simulink library "ride_lib"  (R2025b)
settings: Solver=VariableStepAuto  StartTime=0.0  StopTime=10.0  RelTol=1e-3
undefined symbols (not defined in the file or in its folder): ride
libraries: $bdroot x3
settings Model: Creator=mohammedazab  LastModifiedBy=mohammedazab

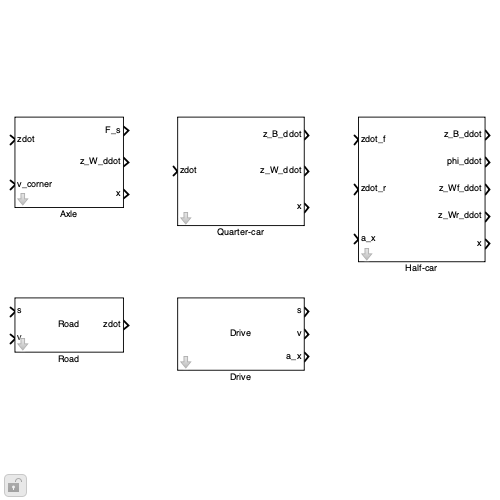
[thumbnail: Simulink's stored preview of the top-level diagram]
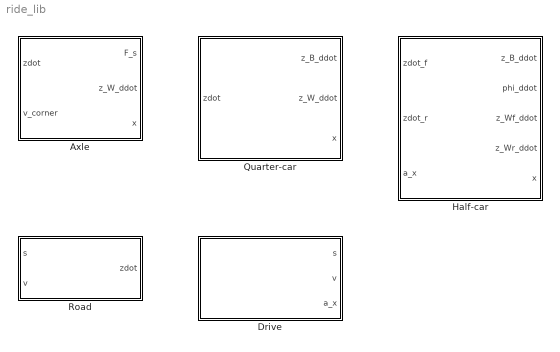
== system ride_lib ==
  Axle : Subsystem  mask(Axle){m_W=50.399999999999999, k_T=262200, c_T=500, k_S=27922, dz_S_stat=0.16361711195473103, dz_cmp=0.02, dz_rbd=0.080000000000000002, f1_cmp=0.33333333329999998, f2_cmp=4, f1_rbd=1, f2_rbd=8, F_max=100000, D=3530, A=0.5, v_d=0.20000000000000001, v_z=0.20000000000000001}
      mask prompts: m_W "Wheel mass m_W [kg]"; k_T "Tyre stiffness k_T [N/m]"; c_T "Tyre damping c_T [N s/m]"; k_S "Spring stiffness k_S [N/m]"; dz_S_stat "Static spring deflection dz_S_stat [m]"; dz_cmp "Compression knee dz_cmp [m]"; dz_rbd "Rebound knee dz_rbd [m]"; f1_cmp "Compression shape f1_cmp [-]"; f2_cmp "Compression rate f2_cmp [-]"; f1_rbd "Rebound shape f1_rbd [-]"; f2_rbd "Rebound rate f2_rbd [-]"; F_max "Spring force limit F_max [N]"; D "Damper coefficient D [N s/m]"; A "Damper asymmetry A [-]"; v_d "Compression knee velocity v_d [m/s]"; v_z "Rebound knee velocity v_z [m/s]"
      mask help: One axle: tyre spring and damper, wheel mass, progressive suspension spring and asymmetric damper. F_s is the suspension force on the body, positive upward. x = [tyre deflection; wheel velocity; suspension deflection].
      mask init:
      | c = ride.core.suspension.damper_coefficients(D, A); d1 = c.d1; z1 = c.z1; d2 = c.d2; z2 = c.z2;
      mask Display:
      | port_label('input', 1, 'zdot');
      | port_label('input', 2, 'v_corner');
      | port_label('output', 1, 'F_s');
      | port_label('output', 2, 'z_W_ddot');
      | port_label('output', 3, 'x');
  Drive : Subsystem  mask(Drive){speeds=6 * ones(500, 1), dt=0.02}
      mask prompts: speeds "Speed at every step [m/s]"; dt "Step dt [s]"
      mask help: Speed profile played back in steps of dt: speed v [m/s] held over each step, distance s [m] and the longitudinal acceleration a_x = (v_k - v_(k-1)) / dt [m/s^2], as in ride.simulate.
      mask init:
      | speed_table = [(0:numel(speeds) - 1)' * dt, speeds(:)];
      mask Display:
      | disp('Drive');
      | port_label('output', 1, 's');
      | port_label('output', 2, 'v');
      | port_label('output', 3, 'a_x');
  Half-car : Subsystem  mask(Half-car){m_B=803, I_B=1430, l_f=1.206, l_r=1.6639999999999999, h_T=0.59999999999999998, h_B=0.222, front_m_W=50.399999999999999, front_k_T=262200, front_c_T=500, front_k_S=29589.900000000001, front_dz_S_stat=0.16361320259798129, front_dz_cmp=0.02, front_dz_rbd=0.080000000000000002, front_f1_cmp=0.33333333329999998, front_f2_cmp=4, front_f1_rbd=1, front_f2_rbd=8, front_F_max=100000, front_D=564.80000000000007, front_A=0.5, front_v_d=0.20000000000000001, front_v_z=0.20000000000000001, rear_m_W=50.399999999999999, rear_k_T=262200, rear_c_T=500, rear_k_S=21444.860000000001, rear_dz_S_stat=0.16361857789913259, rear_dz_cmp=0.02, rear_dz_rbd=0.080000000000000002, rear_f1_cmp=0.33333333329999998, rear_f2_cmp=4, rear_f1_rbd=1, rear_f2_rbd=8, rear_F_max=100000, rear_D=562.39999999999998, rear_A=0.5, rear_v_d=0.20000000000000001, rear_v_z=0.20000000000000001}
      mask prompts: m_B "Body mass m_B [kg]"; I_B "Pitch inertia I_B [kg m^2]"; l_f "Centre of mass to front axle l_f [m]"; l_r "Centre of mass to rear axle l_r [m]"; h_T "Pitch centre height under traction h_T [m]"; h_B "Pitch centre height under braking h_B [m]"; front_m_W "Wheel mass m_W [kg]"; front_k_T "Tyre stiffness k_T [N/m]"; front_c_T "Tyre damping c_T [N s/m]"; front_k_S "Spring stiffness k_S [N/m]"; front_dz_S_stat "Static spring deflection dz_S_stat [m]"; front_dz_cmp "Compression knee dz_cmp [m]"; front_dz_rbd "Rebound knee dz_rbd [m]"; front_f1_cmp "Compression shape f1_cmp [-]"; front_f2_cmp "Compression rate f2_cmp [-]"; front_f1_rbd "Rebound shape f1_rbd [-]"; front_f2_rbd "Rebound rate f2_rbd [-]"; front_F_max "Spring force limit F_max [N]"; front_D "Damper coefficient D [N s/m]"; front_A "Damper asymmetry A [-]"; front_v_d "Compression knee velocity v_d [m/s]"; front_v_z "Rebound knee velocity v_z [m/s]"; rear_m_W "Wheel mass m_W [kg]"; rear_k_T "Tyre stiffness k_T [N/m]"; rear_c_T "Tyre damping c_T [N s/m]"; rear_k_S "Spring stiffness k_S [N/m]"; rear_dz_S_stat "Static spring deflection dz_S_stat [m]"; rear_dz_cmp "Compression knee dz_cmp [m]"; rear_dz_rbd "Rebound knee dz_rbd [m]"; rear_f1_cmp "Compression shape f1_cmp [-]"; rear_f2_cmp "Compression rate f2_cmp [-]"; rear_f1_rbd "Rebound shape f1_rbd [-]"; rear_f2_rbd "Rebound rate f2_rbd [-]"; rear_F_max "Spring force limit F_max [N]"; rear_D "Damper coefficient D [N s/m]"; rear_A "Damper asymmetry A [-]"; rear_v_d "Compression knee velocity v_d [m/s]"; rear_v_z "Rebound knee velocity v_z [m/s]"
      mask help: Half-car ride model: two axles, body heave and pitch, load transfer from the longitudinal acceleration a_x (pitch centre at h_T when a_x > 0, at h_B otherwise). Inputs: road height rate under the front and the rear wheel [m/s] and a_x [m/s^2]. Outputs: body heave and pitch acceleration, front and rear wheel acceleration, and x = [rear tyre deflection; rear wheel velocity; rear suspension deflection; front tyre deflection; front wheel velocity; front suspension deflection; body velocity; pitch rate; body position; pitch angle]. Defaults come from data/models/halfcar/params.json.
      mask init:
      | m_tot = m_B + front_m_W + rear_m_W;
      mask DialogControl body_group Prompt: Body
      mask DialogControl front_group Prompt: Front axle
      mask DialogControl rear_group Prompt: Rear axle
      mask Display:
      | port_label('input', 1, 'zdot_f');
      | port_label('input', 2, 'zdot_r');
      | port_label('input', 3, 'a_x');
      | port_label('output', 1, 'z_B_ddot');
      | port_label('output', 2, 'phi_ddot');
      | port_label('output', 3, 'z_Wf_ddot');
      | port_label('output', 4, 'z_Wr_ddot');
      | port_label('output', 5, 'x');
  Quarter-car : Subsystem  mask(Quarter-car){m_B=465.69999999999999, m_W=50.399999999999999, k_T=262200, c_T=500, k_S=27922, dz_S_stat=0.16361711195473103, dz_cmp=0.02, dz_rbd=0.080000000000000002, f1_cmp=0.33333333329999998, f2_cmp=4, f1_rbd=1, f2_rbd=8, F_max=100000, D=3530, A=0.5, v_d=0.20000000000000001, v_z=0.20000000000000001}
      mask prompts: m_B "Body mass m_B [kg]"; m_W "Wheel mass m_W [kg]"; k_T "Tyre stiffness k_T [N/m]"; c_T "Tyre damping c_T [N s/m]"; k_S "Spring stiffness k_S [N/m]"; dz_S_stat "Static spring deflection dz_S_stat [m]"; dz_cmp "Compression knee dz_cmp [m]"; dz_rbd "Rebound knee dz_rbd [m]"; f1_cmp "Compression shape f1_cmp [-]"; f2_cmp "Compression rate f2_cmp [-]"; f1_rbd "Rebound shape f1_rbd [-]"; f2_rbd "Rebound rate f2_rbd [-]"; F_max "Spring force limit F_max [N]"; D "Damper coefficient D [N s/m]"; A "Damper asymmetry A [-]"; v_d "Compression knee velocity v_d [m/s]"; v_z "Rebound knee velocity v_z [m/s]"
      mask help: Quarter-car ride model: one axle under a quarter of the body, heave only. Input: road height rate under the wheel [m/s]. Outputs: body and wheel vertical acceleration [m/s^2] and the states x = [tyre deflection; wheel velocity; suspension deflection; body velocity; body position]. Defaults come from data/models/quartercar/params.json.
      mask DialogControl body_group Prompt: Body
      mask DialogControl axle_group Prompt: Axle
      mask Display:
      | port_label('input', 1, 'zdot');
      | port_label('output', 1, 'z_B_ddot');
      | port_label('output', 2, 'z_W_ddot');
      | port_label('output', 3, 'x');
  Road : Subsystem  mask(Road){road=ride.core.terrain.bumps([20 0.06 2]), lag_m=0}
      mask prompts: road "Terrain struct (scenario.road)"; lag_m "Distance behind the front axle [m]"
      mask help: Road height rate under a wheel that runs lag_m behind the front axle. road is a terrain struct from ride.core.terrain (a scenario's road field): a bump list or a measured profile.
      mask init:
      | lag = lag_m;
      | if strcmp(road.type, 'profile')
      |     kind = 2; ds = road.ds; dz = road.dz(:); bumps = zeros(1, 3);
      | else
      |     kind = 1; ds = 1; dz = zeros(2, 1); bumps = road.bumps;
      |     if isempty(bumps)
      |         bumps = zeros(1, 3);
      |     end
      | end
      mask Display:
      | disp('Road');
      | port_label('input', 1, 's');
      | port_label('input', 2, 'v');
      | port_label('output', 1, 'zdot');

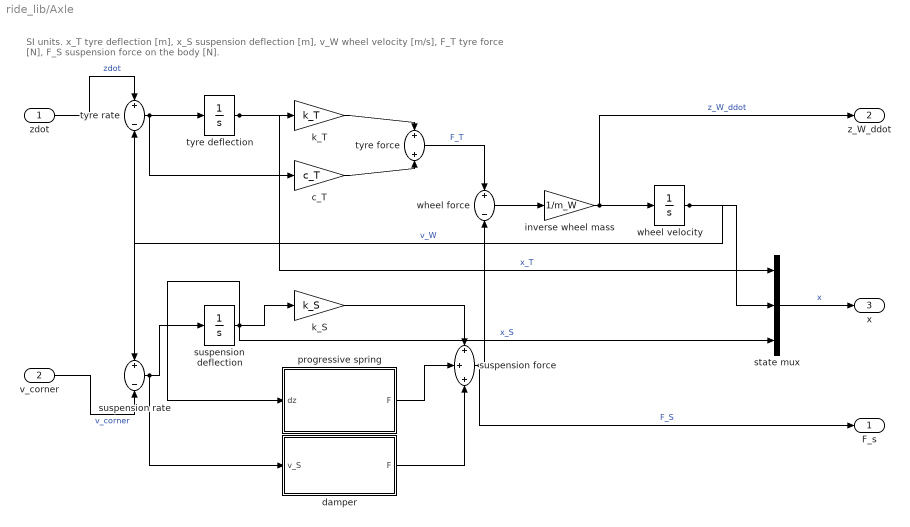
== system ride_lib/Axle ==
  note: SI units. x_T tyre deflection [m], x_S suspension deflection [m], v_W wheel velocity [m/s], F_T tyre force [N], F_S suspension force on the body [N].
  zdot : Inport
  v_corner : Inport  Port=2
  c_T : Gain  Gain=c_T
  damper : MATLAB Function  TreatAsAtomicUnit=on
  inverse wheel mass : Gain  Gain=1/m_W
  k_S : Gain  Gain=k_S
  k_T : Gain  Gain=k_T
  progressive spring : MATLAB Function  TreatAsAtomicUnit=on
  state mux : Mux  Inputs=3
  suspension deflection : Integrator
  suspension force : Sum  Inputs=+++
  suspension rate : Sum  Inputs=+-
  tyre deflection : Integrator
  tyre force : Sum
  tyre rate : Sum  Inputs=+-
  wheel force : Sum  Inputs=+-
  wheel velocity : Integrator
  F_s : Outport
  z_W_ddot : Outport  Port=2
  x : Outport  Port=3
  wires:
  zdot/1 -> tyre rate/1  "zdot"
  wheel velocity/1 -> tyre rate/2, suspension rate/1, state mux/2  "v_W"
  tyre rate/1 -> tyre deflection/1, c_T/1
  tyre deflection/1 -> k_T/1, state mux/1  "x_T"
  k_T/1 -> tyre force/1
  c_T/1 -> tyre force/2
  tyre force/1 -> wheel force/1  "F_T"
  suspension force/1 -> wheel force/2, F_s/1  "F_S"
  wheel force/1 -> inverse wheel mass/1
  inverse wheel mass/1 -> wheel velocity/1, z_W_ddot/1  "z_W_ddot"
  v_corner/1 -> suspension rate/2  "v_corner"
  suspension rate/1 -> suspension deflection/1, damper/1(v_S)
  suspension deflection/1 -> k_S/1, progressive spring/1(dz), state mux/3  "x_S"
  k_S/1 -> suspension force/1
  progressive spring/1(F) -> suspension force/2
  damper/1(F) -> suspension force/3
  state mux/1 -> x/1  "x"

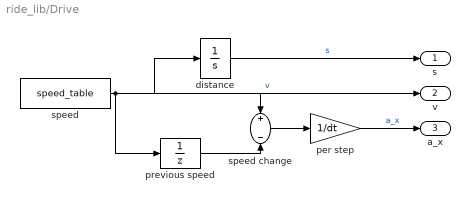
== system ride_lib/Drive ==
  distance : Integrator
  per step : Gain  Gain=1/dt
  previous speed : UnitDelay  InitialCondition=speeds(1)  SampleTime=dt  HasFrameUpgradeWarning=on
  speed : FromWorkspace  VariableName=speed_table  SampleTime=dt  Interpolate=off  OutputAfterFinalValue=Holding final value
  speed change : Sum  Inputs=+-
  s : Outport
  v : Outport  Port=2
  a_x : Outport  Port=3
  wires:
  speed/1 -> distance/1, v/1, speed change/1, previous speed/1  "v"
  distance/1 -> s/1  "s"
  previous speed/1 -> speed change/2
  speed change/1 -> per step/1
  per step/1 -> a_x/1  "a_x"

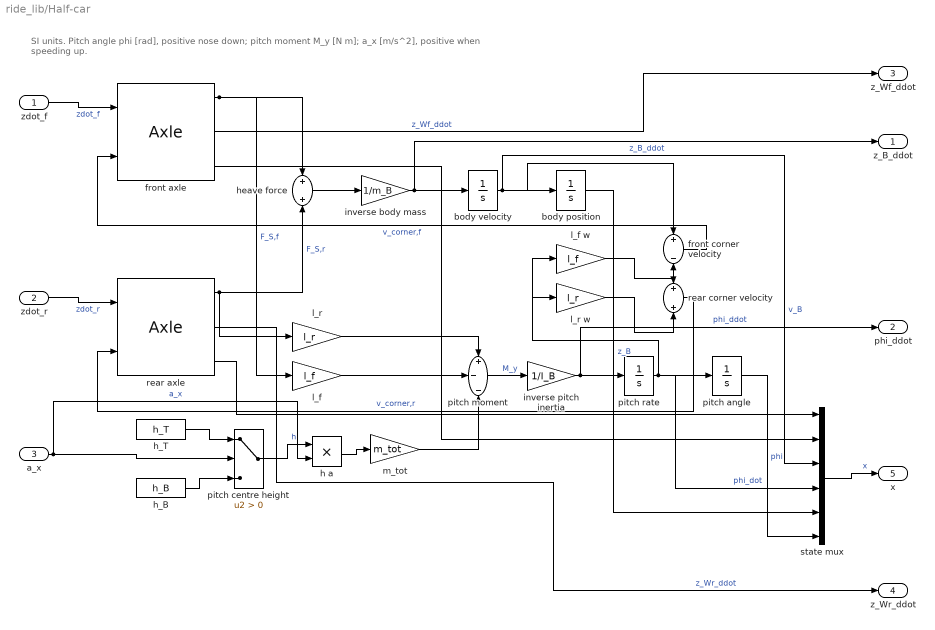
== system ride_lib/Half-car ==
  note: SI units. Pitch angle phi [rad], positive nose down; pitch moment M_y [N m]; a_x [m/s^2], positive when speeding up.
  zdot_f : Inport
  zdot_r : Inport  Port=2
  a_x : Inport  Port=3
  body position : Integrator
  body velocity : Integrator
  front axle : $bdroot/Axle  m_W=front_m_W  k_T=front_k_T  c_T=front_c_T  k_S=front_k_S  dz_S_stat=front_dz_S_stat  dz_cmp=front_dz_cmp  dz_rbd=front_dz_rbd  f1_cmp=front_f1_cmp  f2_cmp=front_f2_cmp  f1_rbd=front_f1_rbd  f2_rbd=front_f2_rbd  F_max=front_F_max  D=front_D  A=front_A  v_d=front_v_d  v_z=front_v_z
  front corner velocity : Sum  Inputs=+-
  h a : Product
  h_B : Constant  Value=h_B
  h_T : Constant  Value=h_T
  heave force : Sum
  inverse body mass : Gain  Gain=1/m_B
  inverse pitch inertia : Gain  Gain=1/I_B
  l_f : Gain  Gain=l_f
  l_f w : Gain  Gain=l_f
  l_r : Gain  Gain=l_r
  l_r w : Gain  Gain=l_r
  m_tot : Gain  Gain=m_tot
  pitch angle : Integrator
  pitch centre height : Switch  Criteria=u2 > Threshold  SaturateOnIntegerOverflow=off  InputSameDT=off
  pitch moment : Sum  Inputs=+--
  pitch rate : Integrator
  rear axle : $bdroot/Axle  m_W=rear_m_W  k_T=rear_k_T  c_T=rear_c_T  k_S=rear_k_S  dz_S_stat=rear_dz_S_stat  dz_cmp=rear_dz_cmp  dz_rbd=rear_dz_rbd  f1_cmp=rear_f1_cmp  f2_cmp=rear_f2_cmp  f1_rbd=rear_f1_rbd  f2_rbd=rear_f2_rbd  F_max=rear_F_max  D=rear_D  A=rear_A  v_d=rear_v_d  v_z=rear_v_z
  rear corner velocity : Sum
  state mux : Mux  Inputs=[3 3 1 1 1 1]
  z_B_ddot : Outport
  phi_ddot : Outport  Port=2
  z_Wf_ddot : Outport  Port=3
  z_Wr_ddot : Outport  Port=4
  x : Outport  Port=5
  wires:
  zdot_f/1 -> front axle/1  "zdot_f"
  zdot_r/1 -> rear axle/1  "zdot_r"
  front corner velocity/1 -> front axle/2  "v_corner,f"
  rear corner velocity/1 -> rear axle/2  "v_corner,r"
  front axle/1 -> heave force/1, l_f/1  "F_S,f"
  rear axle/1 -> heave force/2, l_r/1  "F_S,r"
  heave force/1 -> inverse body mass/1
  inverse body mass/1 -> body velocity/1, z_B_ddot/1  "z_B_ddot"
  body velocity/1 -> body position/1, front corner velocity/1, rear corner velocity/1, state mux/3  "v_B"
  h_T/1 -> pitch centre height/1
  a_x/1 -> pitch centre height/2, h a/2  "a_x"
  h_B/1 -> pitch centre height/3
  pitch centre height/1 -> h a/1  "h"
  h a/1 -> m_tot/1
  l_r/1 -> pitch moment/1
  l_f/1 -> pitch moment/2
  m_tot/1 -> pitch moment/3
  pitch moment/1 -> inverse pitch inertia/1  "M_y"
  inverse pitch inertia/1 -> pitch rate/1, phi_ddot/1  "phi_ddot"
  pitch rate/1 -> pitch angle/1, l_f w/1, l_r w/1, state mux/4  "phi_dot"
  l_f w/1 -> front corner velocity/2
  l_r w/1 -> rear corner velocity/2
  front axle/2 -> z_Wf_ddot/1  "z_Wf_ddot"
  rear axle/2 -> z_Wr_ddot/1  "z_Wr_ddot"
  rear axle/3 -> state mux/1
  front axle/3 -> state mux/2
  body position/1 -> state mux/5  "z_B"
  pitch angle/1 -> state mux/6  "phi"
  state mux/1 -> x/1  "x"

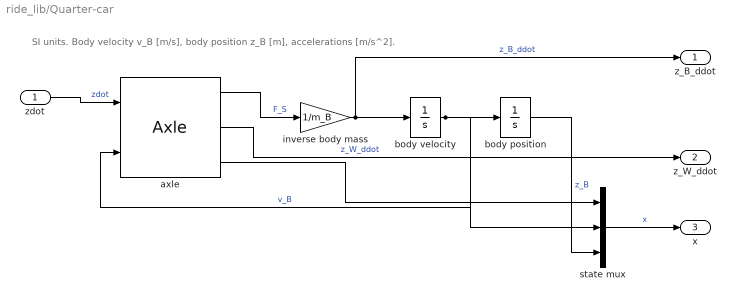
== system ride_lib/Quarter-car ==
  note: SI units. Body velocity v_B [m/s], body position z_B [m], accelerations [m/s^2].
  zdot : Inport
  axle : $bdroot/Axle  m_W=m_W  k_T=k_T  c_T=c_T  k_S=k_S  dz_S_stat=dz_S_stat  dz_cmp=dz_cmp  dz_rbd=dz_rbd  f1_cmp=f1_cmp  f2_cmp=f2_cmp  f1_rbd=f1_rbd  f2_rbd=f2_rbd  F_max=F_max  D=D  A=A  v_d=v_d  v_z=v_z
  body position : Integrator
  body velocity : Integrator
  inverse body mass : Gain  Gain=1/m_B
  state mux : Mux  Inputs=[3 1 1]
  z_B_ddot : Outport
  z_W_ddot : Outport  Port=2
  x : Outport  Port=3
  wires:
  zdot/1 -> axle/1  "zdot"
  body velocity/1 -> axle/2, body position/1, state mux/2  "v_B"
  axle/1 -> inverse body mass/1  "F_S"
  inverse body mass/1 -> body velocity/1, z_B_ddot/1  "z_B_ddot"
  axle/2 -> z_W_ddot/1  "z_W_ddot"
  axle/3 -> state mux/1
  body position/1 -> state mux/3  "z_B"
  state mux/1 -> x/1  "x"

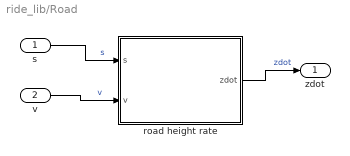
== system ride_lib/Road ==
  s : Inport
  v : Inport  Port=2
  road height rate : MATLAB Function  TreatAsAtomicUnit=on
  zdot : Outport
  wires:
  s/1 -> road height rate/1(s)  "s"
  v/1 -> road height rate/2(v)  "v"
  road height rate/1(zdot) -> zdot/1  "zdot"

== matlab function ride_lib/Axle/damper ==
  data: v_S input; F output; d1 parameter; z1 parameter; d2 parameter; z2 parameter; v_d parameter; v_z parameter
function F = damper(v_S, d1, z1, d2, z2, v_d, v_z)
k = 50;
w_cmp = 1 / (1 + exp(-k * v_S));
F_base = (w_cmp * d1 + (1 - w_cmp) * z1) * v_S;
w_hc = 1 / (1 + exp(-k * (v_S - v_d)));
F_hc = w_hc * (d2 - d1) * (v_S - v_d);
w_hr = 1 / (1 + exp(-k * (-v_S - v_z)));
F_hr = w_hr * (z2 - z1) * (-v_S - v_z);
F = F_base + F_hc - F_hr;
end

== matlab function ride_lib/Axle/progressive spring ==
  data: dz input; F output; k_S parameter; dz_S_stat parameter; dz_cmp parameter; dz_rbd parameter; f1_cmp parameter; f2_cmp parameter; f1_rbd parameter; f2_rbd parameter; F_max parameter
function F = progressive_spring(dz, k_S, dz_S_stat, dz_cmp, dz_rbd, f1_cmp, f2_cmp, f1_rbd, f2_rbd, F_max)
if dz > dz_cmp
    dz_F = dz - dz_cmp;
    F = k_S * (dz_S_stat * f1_cmp * (exp(dz_F * f2_cmp / dz_S_stat) - 1) - dz_F);
elseif dz < -dz_rbd
    dz_F = -dz - dz_rbd;
    F = -k_S * (dz_S_stat * f1_rbd * (exp(dz_F * f2_rbd / dz_S_stat) - 1) - dz_F);
else
    F = 0;
    return
end
F = min(max(F, -F_max), F_max);
end

== matlab function ride_lib/Road/road height rate ==
  data: s input; zdot output; v input; kind parameter; bumps parameter; ds parameter; dz parameter; lag parameter
function zdot = road_height_rate(s, v, kind, bumps, ds, dz, lag)
x = s - lag;
zdot = 0;
if kind == 1
    for i = 1:size(bumps, 1)
        dx = x - bumps(i, 1);
        L = bumps(i, 3);
        if dx > 0 && dx < L
            zdot = (bumps(i, 2) / 2) * (2 * pi / L) * sin(2 * pi * dx / L) * v;
            return
        end
    end
else
    n = numel(dz);
    pos = x / ds;
    if n >= 2 && pos >= 0 && pos <= n - 1
        i = min(floor(pos), n - 2);
        frac = pos - i;
        zdot = (dz(i + 1) * (1 - frac) + dz(i + 2) * frac) * v;
    end
end
end
